simulink model "Servo_ADC"  (Simulink 7.4)
settings: Solver=FixedStepDiscrete  StartTime=0.0  StopTime=10.0  FixedStep=0.001  RelTol=1e-3
undefined symbols (not defined in the file or in its folder): gaind, OC1max, polesd, zerosd
libraries: dsPICdrivers x7
settings Model: Creator=Lubin  LastModifiedBy=Riha9
settings OptimizationCC: InitFltsAndDblsToZero=on  OptimizeModelRefInitCode=on  LifeSpan=1
settings DebuggingCC: SaveWithParameterizedLinksMsg=none  SignalResolutionControl=TryResolveAllWithWarning
settings HardwareCC: ProdBitPerInt=16  ProdEndianess=LittleEndian  ProdWordSize=16  ProdHWDeviceType=16-bit Generic  TargetHWDeviceType=32-bit Generic
settings RTWCC: SystemTargetFile=dspic.tlc  TemplateMakefile=dspic_pic30_gcc.tmf  PostCodeGenCommand=dsPIC_Compile()  Description=Embedded Target for Microchip dsPIC (real-time)  ProcessScript=dspic_make_rtw_hook
settings CodeAppCC: IgnoreCustomStorageClasses=off
settings STFCustomTargetCC: ModelReferenceCompliant=off  IncludeMdlTerminateFcn=off  CombineOutputUpdateFcns=on  SuppressErrorStatus=on  ERTCustomFileBanners=on  SupportContinuousTime=off  SupportNonInlinedSFcns=off  SystemTargetFile=dspic.tlc
settings ERTTargetCC: MultiwordLength=2048  ModelReferenceCompliant=off  ParMdlRefBuildCompliant=off  CompOptLevelCompliant=off  IncludeMdlTerminateFcn=off  SuppressErrorStatus=on  ERTFirstTimeCompliant=off  ModelStepFunctionPrototypeControlCompliant=off  CPPClassGenCompliant=off  InlinedParameterPlacement=NonHierarchical  ERTSrcFileBannerTemplate=dsPIC_code_template.cgt  ERTHdrFileBannerTemplate=dsPIC_code_template.cgt  ERTDataSrcFileTemplate=dsPIC_code_template.cgt  ERTDataHdrFileTemplate=dsPIC_code_template.cgt  ERTCustomFileTemplate=dsPIC_main.tlc  ConvertIfToSwitch=off
settings CustomProperty: DataType=string  Value=C:\PROGRA~1\MATLAB\R2009b\bin\win32\gmake

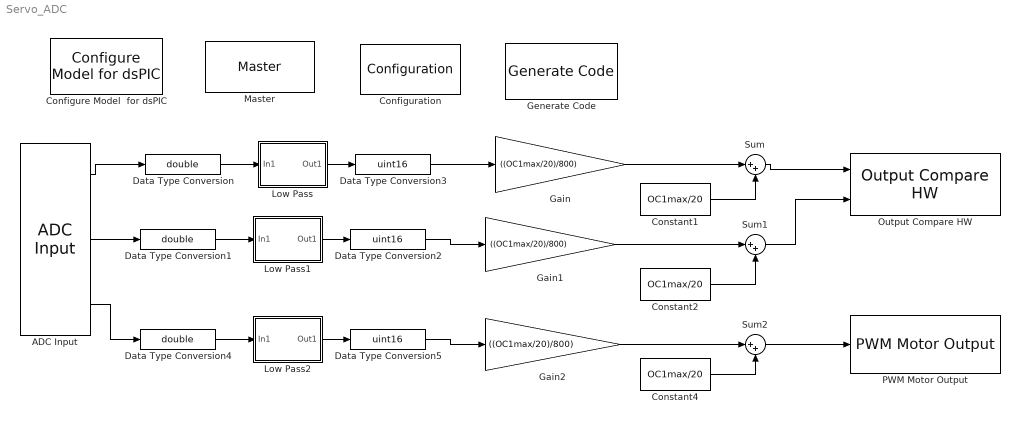
== system Servo_ADC ==
  ADC Input : dsPICdrivers/Peripheral I//O/ADC Input  Tag=dsPIC_ADC  Priority=5  ADC_TYPE=10 bits  ADC_MODE=Continuous sampling & get last channel value  NbrSampleStep=1  VoltRefpopup="AVdd  -  AVss"  OutFormatBitspopup=0000 00dd dddd dddd : Integer  InterruptPriority=3  ANCHANNELS=[2 3 1]  MaxName=ANmax = 1023  Rin=50  ADCS=1  SAMC=1  Temperature=25  DMAChannel=3  SampleTime=-1  Status="OK  |  Tsmp=2.500e-007 |  T/Channel=3.250e-006 |  Tall=9.750e-006"  SSRC=auto convert
  Configuration : dsPICdrivers/Configuration  SystemSampleTime=-1  double64=off
  Configure Model  for dsPIC : dsPICdrivers/Simulink Configuration/Configure Model  for dsPIC
  Constant1 : Constant  Value=OC1max/20  OutDataTypeMode=uint16  OutDataType=sfix(16)  OutScaling=2^0  OutDataTypeStr=uint16
  Constant2 : Constant  Value=OC1max/20  OutDataTypeMode=uint16  OutDataType=sfix(16)  OutScaling=2^0  OutDataTypeStr=uint16
  Constant4 : Constant  Value=OC1max/20  OutDataTypeMode=uint16  OutDataType=sfix(16)  OutScaling=2^0  OutDataTypeStr=uint16
  Data Type Conversion : DataTypeConversion  OutDataTypeMode=double  OutDataType=fixdt(1, 16)  OutScaling=2^0  OutDataTypeStr=double
  Data Type Conversion1 : DataTypeConversion  OutDataTypeMode=double  OutDataType=fixdt(1, 16)  OutScaling=2^0  OutDataTypeStr=double
  Data Type Conversion2 : DataTypeConversion  OutDataTypeMode=uint16  OutDataType=fixdt(1, 16)  OutScaling=2^0  OutDataTypeStr=uint16
  Data Type Conversion3 : DataTypeConversion  OutDataTypeMode=uint16  OutDataType=fixdt(1, 16)  OutScaling=2^0  OutDataTypeStr=uint16
  Data Type Conversion4 : DataTypeConversion  OutDataTypeMode=double  OutDataType=fixdt(1, 16)  OutScaling=2^0  OutDataTypeStr=double
  Data Type Conversion5 : DataTypeConversion  OutDataTypeMode=uint16  OutDataType=fixdt(1, 16)  OutScaling=2^0  OutDataTypeStr=uint16
  Gain : Gain  Gain=((OC1max/20)/800)  ParameterDataType=float('single')  ParameterScaling=2^0  OutDataType=float('single')  OutScaling=2^0
  Gain1 : Gain  Gain=((OC1max/20)/800)  ParameterDataType=float('single')  ParameterScaling=2^0  OutDataType=float('single')  OutScaling=2^0
  Gain2 : Gain  Gain=((OC1max/20)/800)  ParameterDataType=float('single')  ParameterScaling=2^0  OutDataType=float('single')  OutScaling=2^0
  Generate Code : dsPICdrivers/Simulink Configuration/Generate Code
  Low Pass : Subsystem  mask(DiscretizedZeroPole){Zeros=[], Poles=[-15], Gain=15, AbsTol=auto, SampleTime=.01, method=tustin, Wc=1}
      mask prompts: Zeros "Zeros (enter in s-main:)"; Poles "Poles (enter in s-domain:)"; Gain "Gain (enter in s-domain:)"; AbsTol "Absolute tolerance:"; SampleTime "Sample time:"; Wc "Critical Frequency (Hz):"
      mask help: Continuous mask uses c2d to transform parameters onto the Discrete Zero-Pole block inside.
      mask init:
      | st=SampleTime;
      | if length(st)>1
      |     st=SampleTime(1);
      | end
      | if(st>0)
      |     [zerosd,polesd,gaind] = sldiscutil('disczpk', {st,method,Wc,Zeros,Poles,Gain});
      | end	
      | s = get_param(gcb,'maskvalues');
      | zeross = s{1};
      | poless = s{2};
      | gainss = s{3};
      | %zerosc = eval(zeross);
      | %polesc = eval(poless);
      | %gainsc = eval(gainss);
      | sldiscutil('initzpkmask', st);
      | if(st==0)
      | set_param([gcb '/Zero Pole'], 'AbsoluteTolerance', AbsTol);
      | end
      mask StyleString: edit,edit,edit,edit,edit,popup(zoh|foh|tustin|prewarp|matched),edit
      mask CallbackString: |||||hidecrit|
      mask Display:
      | droots(zeross,poless,gainss)
      | text( 0.5, 1.0, method, 'verticalAlignment','top')
  Low Pass1 : Subsystem  mask(DiscretizedZeroPole){Zeros=[], Poles=[-15], Gain=15, AbsTol=auto, SampleTime=.01, method=tustin, Wc=1}
      mask prompts: Zeros "Zeros (enter in s-main:)"; Poles "Poles (enter in s-domain:)"; Gain "Gain (enter in s-domain:)"; AbsTol "Absolute tolerance:"; SampleTime "Sample time:"; Wc "Critical Frequency (Hz):"
      mask help: Continuous mask uses c2d to transform parameters onto the Discrete Zero-Pole block inside.
      mask init: same as Servo_ADC/Low Pass
      mask StyleString: edit,edit,edit,edit,edit,popup(zoh|foh|tustin|prewarp|matched),edit
      mask CallbackString: |||||hidecrit|
      mask Display:
      | droots(zeross,poless,gainss)
      | text( 0.5, 1.0, method, 'verticalAlignment','top')
  Low Pass2 : Subsystem  mask(DiscretizedZeroPole){Zeros=[], Poles=[-15], Gain=15, AbsTol=auto, SampleTime=.01, method=tustin, Wc=1}
      mask prompts: Zeros "Zeros (enter in s-main:)"; Poles "Poles (enter in s-domain:)"; Gain "Gain (enter in s-domain:)"; AbsTol "Absolute tolerance:"; SampleTime "Sample time:"; Wc "Critical Frequency (Hz):"
      mask help: Continuous mask uses c2d to transform parameters onto the Discrete Zero-Pole block inside.
      mask init: same as Servo_ADC/Low Pass
      mask StyleString: edit,edit,edit,edit,edit,popup(zoh|foh|tustin|prewarp|matched),edit
      mask CallbackString: |||||hidecrit|
      mask Display:
      | droots(zeross,poless,gainss)
      | text( 0.5, 1.0, method, 'verticalAlignment','top')
  Master : dsPICdrivers/Master  Tag=dsPIC_MASTER  Priority=1  TimeStepType=Timer1  picType=30f4011  fcy=4e6  Quartz_33f=5e6  PLLActive_33f=off  fcyDesired_33f=0  tmr1="[1  3999  0]"  tmr1Info="Time Step : 0.001  ;   Error : 0%  PR1=3999"  tmr2345="[0  8  0  0]"  tmr2345cfg=[-1 -1 -1 -1]  IOautoConf=on  typePort="[ 0   0   0   0   0   0   0   0   0   0   0   0   0   0   0   0   0   8   8   8   0   0   0   0   0   0   0   0   0   0   0   0   0   0   0   0   0   0   0   0   0   0   0   0   0   0   0   0  24  24  24   0   0   0   0   0   0   0   0   0   0   0   0   0   0   0   0   0   0   0   0   0   0   0   0   0   0   0   0   0   0   0   0   0   0   0   0   0   0   0   0   0   0   0   0   0   0   0   0   0   0   0   0   0   0   0   0   0   0   0   0   0 ]"  TRIS="[ 65535  65535  65535  65528  65535  65535  65535 ]"  ADPCFG=0  MasterBusyPort=None  MasterOverloadPort=None  FOSC=HS  ClockSwitchMonitor=Both disabled  TempProtection_33f=TEMP_ON  FPBOR=PBOR_OFF  PWRT=PWRT_OFF  MCLR=MCLR_EN  ICD=ICS_NONE  JTAGEN=JTAGEN_OFF  PowerSave=off  OverrideFcy=off  NewFcy=1e6  PR2345="[65535   9999  65535  65535]"
  Output Compare HW : dsPICdrivers/Peripheral I//O/Output Compare HW  Tag=dsPIC_OC_HW_out  Priority=5  OC_Mode=PWM duty cycle (robust)  Timer=3  CHANNEL=[1 2]  Channel_UP_Down_Periode="[5  5]"  PeriodeInput=off  MaxChannel=0.02  MaxName=' OCmax '  Precision=[13.2877]  Status=OK  SafeMarge="[0  0]"  PortLetter="[68  68]"  PortNumber="[0  1]"  MaxValues=[9999]  NPORTS=2
  PWM Motor Output : dsPICdrivers/Peripheral I//O/PWM Motor Output  Tag=dsPIC_PWM_Motor  Priority=5  PWMref=1  PWM12=1  InputEnableChk=off  InputPeriodeChk=off  Channel=[1]  TPeriode=.02  PrescalerValue=4  PeriodeInteger=20000  MaxName='PWM'  Centered=off  HChannelON=off  Info="Nbr Bits : 15.2877  ||  PWM = 40000  ||  Prescaler = 4"  Delay=0  IntPriority=5  nbrPwmChannelPIC=3  Status=OK  DeadTimePrescaleA=0  DeadTimePrescaleB=0  DeadTimeInfo=Dead Time A = 0  DTPWM1a=Prescaler A  DTPWM1i=Prescaler A  DTPWM2a=Prescaler A  DTPWM2i=Prescaler A  DTPWM3a=Prescaler A  DTPWM3i=Prescaler A  DTPWM4a=Prescaler A  DTPWM4i=Prescaler A  DTCON1=0  DTCON2=0
  Sum : Sum  Inputs=|++  OutDataTypeMode=uint16  OutDataType=sfix(16)  OutScaling=2^0  OutDataTypeStr=uint16
  Sum1 : Sum  Inputs=|++  OutDataTypeMode=uint16  OutDataType=sfix(16)  OutScaling=2^0  OutDataTypeStr=uint16
  Sum2 : Sum  Inputs=|++  OutDataTypeMode=uint16  OutDataType=sfix(16)  OutScaling=2^0  OutDataTypeStr=uint16
  wires:
  Data Type Conversion/1 -> Low Pass/1(In1)
  Low Pass/1(Out1) -> Data Type Conversion3/1
  Constant1/1 -> Sum/2
  Gain/1 -> Sum/1
  ADC Input/1 -> Data Type Conversion/1
  Data Type Conversion3/1 -> Gain/1
  Data Type Conversion1/1 -> Low Pass1/1(In1)
  Low Pass1/1(Out1) -> Data Type Conversion2/1
  Constant2/1 -> Sum1/2
  Gain1/1 -> Sum1/1
  Data Type Conversion2/1 -> Gain1/1
  ADC Input/2 -> Data Type Conversion1/1
  Sum/1 -> Output Compare HW/1
  Sum1/1 -> Output Compare HW/2
  Data Type Conversion4/1 -> Low Pass2/1(In1)
  Low Pass2/1(Out1) -> Data Type Conversion5/1
  Constant4/1 -> Sum2/2
  Gain2/1 -> Sum2/1
  Data Type Conversion5/1 -> Gain2/1
  ADC Input/3 -> Data Type Conversion4/1
  Sum2/1 -> PWM Motor Output/1

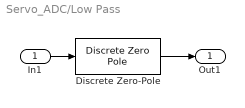
== system Servo_ADC/Low Pass ==
  In1 : Inport  OutDataType=sfix(16)  OutScaling=2^0
  Discrete Zero-Pole : DiscreteZeroPole  Zeros=zerosd  Poles=polesd  Gain=gaind  SampleTime=SampleTime
  Out1 : Outport  OutDataType=sfix(16)  OutScaling=2^0
  wires:
  In1/1 -> Discrete Zero-Pole/1
  Discrete Zero-Pole/1 -> Out1/1

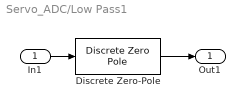
== system Servo_ADC/Low Pass1 ==
  In1 : Inport  OutDataType=sfix(16)  OutScaling=2^0
  Discrete Zero-Pole : DiscreteZeroPole  Zeros=zerosd  Poles=polesd  Gain=gaind  SampleTime=SampleTime
  Out1 : Outport  OutDataType=sfix(16)  OutScaling=2^0
  wires:
  Discrete Zero-Pole/1 -> Out1/1
  In1/1 -> Discrete Zero-Pole/1

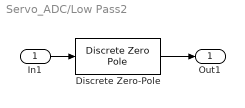
== system Servo_ADC/Low Pass2 ==
  In1 : Inport  OutDataType=sfix(16)  OutScaling=2^0
  Discrete Zero-Pole : DiscreteZeroPole  Zeros=zerosd  Poles=polesd  Gain=gaind  SampleTime=SampleTime
  Out1 : Outport  OutDataType=sfix(16)  OutScaling=2^0
  wires:
  In1/1 -> Discrete Zero-Pole/1
  Discrete Zero-Pole/1 -> Out1/1
